simulink model "six_pulse_thyristor_based_rectifier"  (R2026b)
settings: Solver=ode23tb  StopTime=param.sim.simlength  FixedStep=param.glb_time.tc  MaxStep=param.glb_time.tc  EnableMultiTasking=on
values from neighbouring files (symbols this model uses):
  param = struct()    [init_model.m]    (also in init_model_legacy.m = add_template_extras(param, options))
undefined symbols (not defined in the file or in its folder): magnitude
libraries: fl_lib x168, nesl_utility x52, ee_lib x8, thyristor_rr_lib x6, first_harmonic_tracker x3, three_phase_voltage_with_frt_emulator x1
(part 1 of 4)
settings Model: Creator=LTNBDA  LastModifiedBy=d.bagnara
settings SolverCC: SolverResetMethod=Robust  ZeroCrossAlgorithm=Adaptive  ZeroCrossControl=EnableAll
settings DataIOCC: LimitDataPoints=on  MaxDataPoints=1  ReturnWorkspaceOutputs=off  SaveFormat=Array  SignalLoggingSaveFormat=ModelDataLogs
settings OptimizationCC: EfficientMapNaN2IntZero=off  LifeSpan=inf  MemsetInitFltsAndDblsToZero=off
settings DebuggingCC: ArithmeticOperatorsInVariantConditions=warning  FcnCallInpInsideContextMsg=warning  MergeDetectMultiDrivingBlocksExec=none  MultiTaskCondExecSysMsg=none  MultiTaskDSMMsg=warning  SFNoUnconditionalDefaultTransitionDiag=warning  SFUnexpectedBacktrackingDiag=warning  SaveWithParameterizedLinksMsg=none  SignalResolutionControl=TryResolveAllWithWarning  SolverPrmCheckMsg=warning  StateNameClashWarn=warning
settings HardwareCC: ProdEndianess=Unspecified  ProdEqTarget=off  ProdHWDeviceType=Generic->64-bit Embedded Processor (LP64)  ProdIntDivRoundTo=Undefined  ProdLargestAtomicFloat=None  TargetEndianess=LittleEndian  TargetHWDeviceType=MATLAB Host  TargetIntDivRoundTo=Zero  TargetLongLongMode=on
settings ModelReferenceCC: PropagateSignalLabelsOutOfModel=off
settings SFSimCC: CustomCodeUndefinedFunction=UseInterfaceOnly  SimUseLocalCustomCode=off
settings SFSimCC: SimCustomHeaderCode=|
  | #include "math_f.h"
  | #include "mavgflt.h"
  | #include "mavgflt_simulink.h"
  | #include "bemf_obsv.h"
  | #include "bemf_obsv_simulink.h"
  | #include "bemf_obsv_load_est.h"
  | #include "bemf_obsv_load_est_simulink.h"
  | #include "dqvector_pi.h"
  | #include "dqvector_pi_simulink.h"
  | #include "sv_pwm_simulink.h"
  | #include "sv_pwm.h"
  | #include "six_pulse_rect.h"
  | #include "twelve_pulse_rect.h"
  | #include "first_harmonic_tracker.h"
  | #include "first_harmonic_tracker_simulink.h"
  | #include "dqpll_thyr.h"
  | #include "dqpll_thyr_simulink.h"
  | #include "dqpll_grid.h"
  | #include "dqpll_grid_simulink.h"
settings SFSimCC: SimUserIncludeDirs=|
  | include
  | src
settings SFSimCC: SimUserSources=|
  | "mavgflt_simulink.c"
  | "mavgflt.c"
  | "bemf_obsv_simulink.c"
  | "bemf_obsv.c"
  | "bemf_obsv_load_est_simulink.c"
  | "bemf_obsv_load_est.c"
  | "dqvector_pi.c"
  | "dqvector_pi_simulink.c"
  | "sv_pwm_simulink.c"
  | "sv_pwm.c"
  | "six_pulse_rect.c"
  | "twelve_pulse_rect.c"
  | "first_harmonic_tracker_simulink.c"
  | "first_harmonic_tracker.c"
  | "dqpll_thyr_simulink.c"
  | "dqpll_thyr.c"
  | "dqpll_grid_simulink.c"
  | "dqpll_grid.c"
settings RTWCC: RTWUseLocalCustomCode=off
settings CodeAppCC: StateflowObjectComments=on
settings GRTTargetCC: CombineOutputUpdateFcns=off  GRTInterface=on  TargetLangStandard=C89/C90 (ANSI)
settings ConfigComp: CovExternalEMLEnable=off  CovSaveCumulativeToWorkspaceVar=on  CovSaveSingleToWorkspaceVar=on
settings SimscapeCC: SimscapeNormalizeSystem=off  SimscapeUseEnergyAccounting=off

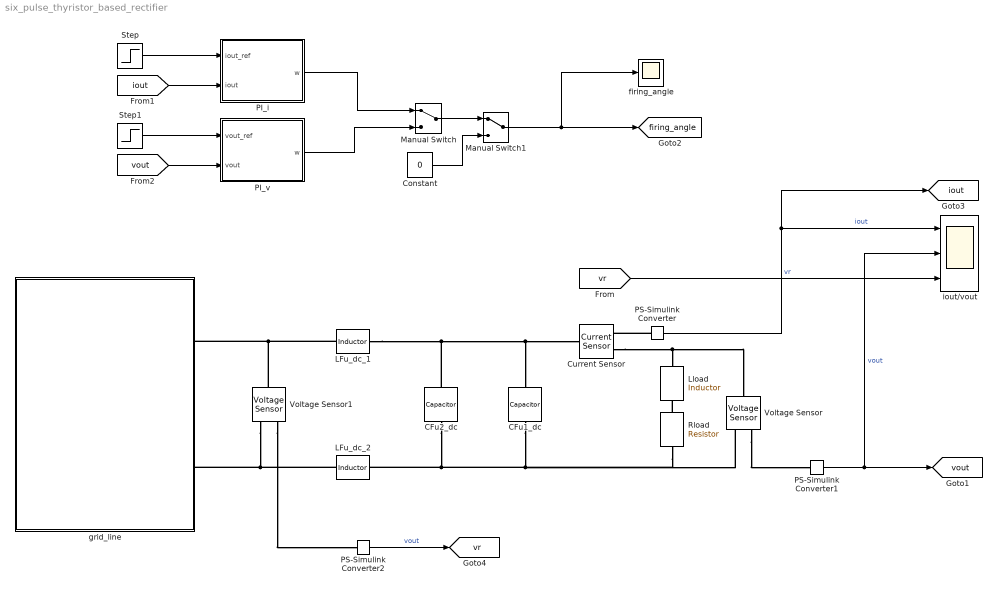
== system six_pulse_thyristor_based_rectifier ==
  CFu1_dc : fl_lib/Electrical/Electrical Elements/Capacitor  c=param.rect.hw.CFu1_dc F  r=param.rect.hw.RCFu1_dc Ohm  g=0 1/Ohm  i_specify=off  i_priority=None  i=0 A  i_nominal_specify=off  i_nominal_value=1  i_nominal_unit=A  v_specify=off  v_priority=None  v=0 V  v_nominal_specify=off  v_nominal_value=1  v_nominal_unit=V  vc_specify=off  vc_priority=High  vc=0 V  vc_nominal_specify=off  vc_nominal_value=1  vc_nominal_unit=V
  CFu2_dc : fl_lib/Electrical/Electrical Elements/Capacitor  c=param.rect.hw.CFu2_dc F  r=param.rect.hw.RCFu2_dc Ohm  g=0 1/Ohm  i_specify=off  i_priority=None  i=0 A  i_nominal_specify=off  i_nominal_value=1  i_nominal_unit=A  v_specify=off  v_priority=None  v=0 V  v_nominal_specify=off  v_nominal_value=1  v_nominal_unit=V  vc_specify=off  vc_priority=High  vc=0 V  vc_nominal_specify=off  vc_nominal_value=1  vc_nominal_unit=V
  Constant : Constant  Value=0
  Current Sensor : fl_lib/Electrical/Electrical Sensors/Current Sensor
  LFu_dc_1 : fl_lib/Electrical/Electrical Elements/Inductor  l=param.rect.hw.LFu_dc/2 H  r=param.rect.hw.RLFu_dc/2 Ohm  g=1e-9 1/Ohm  i_specify=off  i_priority=None  i=0 A  i_nominal_specify=off  i_nominal_value=1  i_nominal_unit=A  v_specify=off  v_priority=None  v=0 V  v_nominal_specify=off  v_nominal_value=1  v_nominal_unit=V  i_L_specify=off  i_L_priority=High  i_L=0 A  i_L_nominal_specify=off  i_L_nominal_value=1  i_L_nominal_unit=A
  LFu_dc_2 : fl_lib/Electrical/Electrical Elements/Inductor  l=param.rect.hw.LFu_dc/2 H  r=param.rect.hw.RLFu_dc/2 Ohm  g=1e-9 1/Ohm  i_specify=off  i_priority=None  i=0 A  i_nominal_specify=off  i_nominal_value=1  i_nominal_unit=A  v_specify=off  v_priority=None  v=0 V  v_nominal_specify=off  v_nominal_value=1  v_nominal_unit=V  i_L_specify=off  i_L_priority=High  i_L=0 A  i_L_nominal_specify=off  i_L_nominal_value=1  i_L_nominal_unit=A
  Lload : fl_lib/Electrical/Electrical Elements/Inductor  l=param.load.L H  r=0 Ohm  g=1e-9 1/Ohm  i_specify=off  i_priority=None  i=0 A  i_nominal_specify=off  i_nominal_value=1  i_nominal_unit=A  v_specify=off  v_priority=None  v=0 V  v_nominal_specify=off  v_nominal_value=1  v_nominal_unit=V  i_L_specify=off  i_L_priority=High  i_L=0 A  i_L_nominal_specify=off  i_L_nominal_value=1  i_L_nominal_unit=A
  Manual Switch : ManualSwitch
  Manual Switch1 : ManualSwitch
  PI_i : Subsystem
  PI_v : Subsystem
  PS-Simulink Converter : nesl_utility/PS-Simulink Converter  PhysicalDomain=network_engine_domain  SubClassName=ps_output  LeftPortType=input  RightPortType=output  PseudoPeriodic=off  Frequencies=[]  VectorFormat=1-D array  Unit=A  AffineConversion=off
  PS-Simulink Converter1 : nesl_utility/PS-Simulink Converter  PhysicalDomain=network_engine_domain  SubClassName=ps_output  LeftPortType=input  RightPortType=output  PseudoPeriodic=off  Frequencies=[]  VectorFormat=1-D array  Unit=V  AffineConversion=on
  PS-Simulink Converter2 : nesl_utility/PS-Simulink Converter  PhysicalDomain=network_engine_domain  SubClassName=ps_output  LeftPortType=input  RightPortType=output  PseudoPeriodic=off  Frequencies=[]  VectorFormat=1-D array  Unit=V  AffineConversion=on
  Rload : fl_lib/Electrical/Electrical Elements/Resistor  R=param.load.R Ohm  i_specify=off  i_priority=None  i=0 A  i_nominal_specify=off  i_nominal_value=1  i_nominal_unit=A  v_specify=off  v_priority=None  v=0 V  v_nominal_specify=off  v_nominal_value=1  v_nominal_unit=V
  Step : Step  Time=param.rect.ctrl.t_iref_step  InitialValue=param.rect.ctrl.iref_1/param.meas.I_FS  FinalValue=param.rect.ctrl.iref_2/param.meas.I_FS  SampleTime=0
  Step1 : Step  Time=0  FinalValue=param.rect.ctrl.vref/param.meas.V_FS  SampleTime=0
  Voltage Sensor : fl_lib/Electrical/Electrical Sensors/Voltage Sensor
  Voltage Sensor1 : fl_lib/Electrical/Electrical Sensors/Voltage Sensor
  firing_angle : Scope
      settings: ActiveDisplayYMinimum=-0.39269908169872403  ActiveDisplayYMaximum=3.5342917352885173  DataLoggingVariableName=ScopeData5
  grid_line : Subsystem
  iout/vout : Scope  NumInputPorts=3
      settings: ActiveDisplayYMinimum=-22.431866208860185  ActiveDisplayYMaximum=201.8867958797417  DataLoggingVariableName=ScopeData10
  tag scope: firing_angle=global, iout=global, vout=global, vr=global
  wires:
  PS-Simulink Converter/1 -> [iout], iout/vout/1  "iout"
  Step/1 -> PI_i/1(iout_ref)
  PS-Simulink Converter1/1 -> [vout], iout/vout/2  "vout"
  [iout] -> PI_i/2(iout)
  [vout] -> PI_v/2(vout)
  Step1/1 -> PI_v/1(vout_ref)
  PI_i/1(w) -> Manual Switch/1
  PI_v/1(w) -> Manual Switch/2
  Manual Switch/1 -> Manual Switch1/1
  Manual Switch1/1 -> [firing_angle], firing_angle/1
  Constant/1 -> Manual Switch1/2
  PS-Simulink Converter2/1 -> [vr]  "vout"
  [vr] -> iout/vout/3  "vr"
  connections:
  LFu_dc_1/RConn1 -- CFu2_dc/LConn1 -- Current Sensor/LConn1 -- CFu1_dc/LConn1
  CFu1_dc/RConn1 -- LFu_dc_2/LConn1 -- CFu2_dc/RConn1 -- Voltage Sensor/RConn2 -- Rload/RConn1
  LFu_dc_2/RConn1 -- Voltage Sensor1/RConn2 -- grid_line/RConn2
  LFu_dc_1/LConn1 -- Voltage Sensor1/LConn1 -- grid_line/RConn1
  Rload/LConn1 -- Lload/RConn1
  PS-Simulink Converter/LConn1 -- Current Sensor/RConn1
  Current Sensor/RConn2 -- Voltage Sensor/LConn1 -- Lload/LConn1
  Voltage Sensor/RConn1 -- PS-Simulink Converter1/LConn1
  Voltage Sensor1/RConn1 -- PS-Simulink Converter2/LConn1

== system six_pulse_thyristor_based_rectifier/PI_i ==
  iout_ref : Inport
  iout : Inport  Port=2
  1/Ti : Gain  Gain=param.rect.ctrl.pi_i.kp  SaturateOnIntegerOverflow=on  OutDataTypeStr=Inherit: Same as input  ParamDataTypeStr=Inherit: Same as input
  1/Ti2 : Gain  Gain=1/param.meas.I_FS  SaturateOnIntegerOverflow=on  OutDataTypeStr=Inherit: Same as input  ParamDataTypeStr=Inherit: Same as input
  Saturation : Saturate  UpperLimit=param.rect.ctrl.alpha_max  LowerLimit=param.rect.ctrl.alpha_min
  Saturation1 : Saturate  UpperLimit=param.rect.ctrl.u_max  LowerLimit=param.rect.ctrl.u_min
  Sum1 : Sum  Inputs=+++  SaturateOnIntegerOverflow=on
  Sum2 : Sum  Inputs=+-  SaturateOnIntegerOverflow=on
  Sum3 : Sum  Inputs=-+  SaturateOnIntegerOverflow=on
  Trigonometric Function : Trigonometry  Operator=acos
  Unit Delay1 : UnitDelay  SampleTime=param.glb_time.ts_rect
  Unit Delay4 : UnitDelay  SampleTime=param.glb_time.ts_rect
  kp : Gain  Gain=param.rect.ctrl.pi_i.ki*param.glb_time.ts_rect  SaturateOnIntegerOverflow=on  OutDataTypeStr=Inherit: Same as input  ParamDataTypeStr=Inherit: Same as input
  tracking_current : Scope  NumInputPorts=2
      settings: ActiveDisplayYMinimum=-0.16727670721082677  ActiveDisplayYMaximum=1.5054903648974411  DataLoggingVariableName=ScopeData7
  w : Outport  VectorParamsAs1DForOutWhenUnconnected=off
  wires:
  Sum2/1 -> 1/Ti/1, kp/1
  kp/1 -> Sum1/2
  1/Ti/1 -> Sum3/1, Sum1/1
  Unit Delay4/1 -> Sum1/3
  Sum3/1 -> Unit Delay4/1
  Sum1/1 -> Saturation1/1
  Saturation/1 -> Unit Delay1/1
  iout/1 -> 1/Ti2/1
  iout_ref/1 -> tracking_current/1, Sum2/1  "i_out_ref"
  1/Ti2/1 -> Sum2/2, tracking_current/2  "i_out"
  Unit Delay1/1 -> w/1
  Saturation1/1 -> Sum3/2, Trigonometric Function/1
  Trigonometric Function/1 -> Saturation/1

== system six_pulse_thyristor_based_rectifier/PI_v ==
  vout_ref : Inport
  vout : Inport  Port=2
  1/Ti : Gain  Gain=param.rect.ctrl.pi_v.kp  SaturateOnIntegerOverflow=on  OutDataTypeStr=Inherit: Same as input  ParamDataTypeStr=Inherit: Same as input
  1/Ti2 : Gain  Gain=1/param.meas.V_FS  SaturateOnIntegerOverflow=on  OutDataTypeStr=Inherit: Same as input  ParamDataTypeStr=Inherit: Same as input
  Saturation : Saturate  UpperLimit=param.rect.ctrl.alpha_max  LowerLimit=param.rect.ctrl.alpha_min
  Saturation1 : Saturate  UpperLimit=param.rect.ctrl.u_max  LowerLimit=param.rect.ctrl.u_min
  Sum1 : Sum  Inputs=+++  SaturateOnIntegerOverflow=on
  Sum2 : Sum  Inputs=+-  SaturateOnIntegerOverflow=on
  Sum3 : Sum  Inputs=-+  SaturateOnIntegerOverflow=on
  Trigonometric Function : Trigonometry  Operator=acos
  Unit Delay1 : UnitDelay  SampleTime=param.glb_time.ts_rect
  Unit Delay4 : UnitDelay  SampleTime=param.glb_time.ts_rect
  kp : Gain  Gain=param.rect.ctrl.pi_v.ki*param.glb_time.ts_rect  SaturateOnIntegerOverflow=on  OutDataTypeStr=Inherit: Same as input  ParamDataTypeStr=Inherit: Same as input
  w : Outport  VectorParamsAs1DForOutWhenUnconnected=off
  wires:
  Trigonometric Function/1 -> Saturation/1
  Saturation1/1 -> Trigonometric Function/1, Sum3/2
  Unit Delay1/1 -> w/1
  1/Ti2/1 -> Sum2/2
  vout_ref/1 -> Sum2/1
  vout/1 -> 1/Ti2/1
  Saturation/1 -> Unit Delay1/1
  Sum1/1 -> Saturation1/1
  Sum3/1 -> Unit Delay4/1
  Unit Delay4/1 -> Sum1/3
  1/Ti/1 -> Sum1/1, Sum3/1
  kp/1 -> Sum1/2
  Sum2/1 -> kp/1, 1/Ti/1

== system six_pulse_thyristor_based_rectifier/grid_line ==
  Grid : Subsystem
  six_pulse rectifier : Subsystem
  DC+ : PMIOPort  Side=Right
  DC- : PMIOPort  Port=2  Side=Right
  connections:
  six_pulse rectifier/RConn1 -- DC+/RConn1
  Grid/RConn1 -- six_pulse rectifier/LConn1
  six_pulse rectifier/RConn2 -- DC-/RConn1

== system six_pulse_thyristor_based_rectifier/grid_line/Grid ==
  Dyg_TR : Subsystem
  grid_emulator : Subsystem
  pwr-measurement : Subsystem
  u_grid : PMIOPort  Side=Right
  connections:
  Dyg_TR/LConn2 -- grid_emulator/RConn2
  Dyg_TR/LConn1 -- grid_emulator/RConn1
  Dyg_TR/LConn3 -- grid_emulator/RConn3
  Dyg_TR/RConn1 -- u_grid/RConn1

== system six_pulse_thyristor_based_rectifier/grid_line/six_pulse rectifier ==
  BR2 : Subsystem
  C-caller ctrl : Subsystem
  Inductor : fl_lib/Electrical/Electrical Elements/Inductor  l=param.rect.hw.Lac H  r=0 Ohm  g=1e-9 1/Ohm  i_specify=off  i_priority=None  i=0 A  i_nominal_specify=off  i_nominal_value=1  i_nominal_unit=A  v_specify=off  v_priority=None  v=0 V  v_nominal_specify=off  v_nominal_value=1  v_nominal_unit=V  i_L_specify=off  i_L_priority=High  i_L=0 A  i_L_nominal_specify=off  i_L_nominal_value=1  i_L_nominal_unit=A
  Inductor1 : fl_lib/Electrical/Electrical Elements/Inductor  l=param.rect.hw.Lac H  r=0 Ohm  g=1e-9 1/Ohm  i_specify=off  i_priority=None  i=0 A  i_nominal_specify=off  i_nominal_value=1  i_nominal_unit=A  v_specify=off  v_priority=None  v=0 V  v_nominal_specify=off  v_nominal_value=1  v_nominal_unit=V  i_L_specify=off  i_L_priority=High  i_L=0 A  i_L_nominal_specify=off  i_L_nominal_value=1  i_L_nominal_unit=A
  Inductor2 : fl_lib/Electrical/Electrical Elements/Inductor  l=param.rect.hw.Lac H  r=0 Ohm  g=1e-9 1/Ohm  i_specify=off  i_priority=None  i=0 A  i_nominal_specify=off  i_nominal_value=1  i_nominal_unit=A  v_specify=off  v_priority=None  v=0 V  v_nominal_specify=off  v_nominal_value=1  v_nominal_unit=V  i_L_specify=off  i_L_priority=High  i_L=0 A  i_L_nominal_specify=off  i_L_nominal_value=1  i_L_nominal_unit=A
  Phase Splitter2 : ee_lib/Connectors & References/Phase Splitter
  Scope2 : Scope
      settings: SampleTime=param.glb_time.ts_rect  ActiveDisplayYMinimum=-0.78504431247711159  ActiveDisplayYMaximum=7.0653988122940063
  Step : Step  Time=param.rect.ctrl.t_pulse_release  InitialValue=1  FinalValue=0  SampleTime=param.glb_time.ts_rect
  pll : Subsystem
  ui/grid : Scope  NumInputPorts=2
      settings: ActiveDisplayYMinimum=-5.4212636300708823  ActiveDisplayYMaximum=7.6356213899946326
  voltage_measure1 : Subsystem
  voltage_measure2 : Subsystem
  DC+ : PMIOPort  Side=Right
  grid_line : PMIOPort  Port=2  Side=Left
  DC- : PMIOPort  Port=3  Side=Right
  wires:
  voltage_measure2/1(vabc_grid) -> ui/grid/1
  Step/1 -> C-caller ctrl/3(Block)
  pll/1(grid_phase_hat) -> Scope2/1, C-caller ctrl/2(wt)
  [firing_angle] -> C-caller ctrl/1(alpha)
  voltage_measure2/2(iabc_grid) -> ui/grid/2
  C-caller ctrl/1(firing_cmds) -> BR2/1(firing_cmds)
  connections:
  voltage_measure2/RConn1 -- BR2/RConn1
  grid_line/RConn1 -- Phase Splitter2/LConn1
  voltage_measure1/LConn2 -- Inductor1/RConn1 -- voltage_measure2/LConn2
  voltage_measure1/LConn3 -- Inductor2/RConn1 -- voltage_measure2/LConn3
  BR2/LConn2 -- DC-/RConn1
  voltage_measure2/RConn3 -- BR2/RConn3
  voltage_measure1/LConn1 -- Inductor/RConn1 -- voltage_measure2/LConn1
  voltage_measure2/RConn2 -- BR2/RConn2
  BR2/LConn1 -- DC+/RConn1
  Phase Splitter2/RConn1 -- Inductor/LConn1
  Phase Splitter2/RConn2 -- Inductor1/LConn1
  Phase Splitter2/RConn3 -- Inductor2/LConn1

== system six_pulse_thyristor_based_rectifier/grid_line/Grid/Dyg_TR ==
  Electrical Reference : fl_lib/Electrical/Electrical Elements/Electrical Reference
  PS Terminator : fl_lib/Physical Signals/Sinks/PS Terminator
  PS Terminator1 : fl_lib/Physical Signals/Sinks/PS Terminator
  PS Terminator2 : fl_lib/Physical Signals/Sinks/PS Terminator
  Phase Splitter : ee_lib/Connectors & References/Phase Splitter
  configurable_trafo : SimscapeComponentBlock  Description=Configurable transformer: one or two three-phase primaries (star or delta), secondary three-phase (star or delta, any clock number) or single-phase (turns distribution ws) on a three-limb core. Component configurable_transformer.configurable_transformer (pwr-control/library, foundation/electrical_machines/+configurable_transformer).  SourceFile=configurable_transformer.configurable_transformer  ComponentPath=configurable_transformer.configurable_transformer  ComponentVariants="[\"configurable_transformer.configurable_transformer\"]"  ComponentVariantNames="[\"configurable_transformer\"]"  ClassName=configurable_transformer  SchemaVersion=1  primaries=configurable_transformer.n_primaries.one  conn1=configurable_transformer.connection.delta  conn2=configurable_transformer.connection.star  clock2=param.grid.trafo.clock2  secondary=configurable_transformer.secondary_winding.star  clock3=param.grid.trafo.clock3  ws=[1, -1, 0]  Sr=param.grid.trafo.Sr A*V  V1=param.grid.trafo.V1 V  V2=param.grid.trafo.V2 V  V3=param.grid.trafo.V3 V  fr=param.grid.trafo.fr Hz  r1=param.grid.trafo.r1  l1=param.grid.trafo.l1  r2=param.grid.trafo.r2  l2=param.grid.trafo.l2  r3=param.grid.trafo.r3  l3=param.grid.trafo.l3  lm=param.grid.trafo.lm  lm0=param.grid.trafo.lm0  rfe=param.grid.trafo.rfe  i1a_specify=off  i1a_priority=None  i1a=0 A  i1a_nominal_specify=off  i1a_nominal_value=1  i1a_nominal_unit=A  i1b_specify=off  i1b_priority=None  i1b=0 A  i1b_nominal_specify=off  i1b_nominal_value=1  i1b_nominal_unit=A  i1c_specify=off  i1c_priority=None  i1c=0 A  i1c_nominal_specify=off  i1c_nominal_value=1  i1c_nominal_unit=A  i2a_specify=off  i2a_priority=None  i2a=0 A  i2a_nominal_specify=off  i2a_nominal_value=1  i2a_nominal_unit=A  i2b_specify=off  i2b_priority=None  i2b=0 A  i2b_nominal_specify=off  i2b_nominal_value=1  i2b_nominal_unit=A  i2c_specify=off  i2c_priority=None  i2c=0 A  i2c_nominal_specify=off  i2c_nominal_value=1  i2c_nominal_unit=A  i3a_specify=off  i3a_priority=None  i3a=0 A  i3a_nominal_specify=off  i3a_nominal_value=1  i3a_nominal_unit=A  i3b_specify=off  i3b_priority=None  i3b=0 A  i3b_nominal_specify=off  i3b_nominal_value=1  i3b_nominal_unit=A  i3c_specify=off  i3c_priority=None  i3c=0 A  i3c_nominal_specify=off  i3c_nominal_value=1  i3c_nominal_unit=A  i3_specify=off  i3_priority=None  i3=0 A  i3_nominal_specify=off  i3_nominal_value=1  i3_nominal_unit=A
      settings: CopyFcn=simscape.sscblock.internal.componentBlockCallback(gcbh,'COPY')  PreCopyFcn=simscape.sscblock.internal.componentBlockCallback(gcbh,'PRECOPY')  PreDeleteFcn=simscape.sscblock.internal.componentBlockCallback(gcbh,'PREDELETE')
      mask Type: Configurable Transformer
  ui_meas : Subsystem
  u1_a : PMIOPort  Side=Left
  u1_b : PMIOPort  Port=2  Side=Left
  u1_c : PMIOPort  Port=3  Side=Left
  u2_abc : PMIOPort  Port=4  Side=Right
  connections:
  configurable_trafo/LConn1 -- u1_a/RConn1
  configurable_trafo/LConn2 -- u1_b/RConn1
  configurable_trafo/LConn3 -- u1_c/RConn1
  configurable_trafo/RConn4 -- Electrical Reference/LConn1
  u2_abc/RConn1 -- Phase Splitter/LConn1
  PS Terminator/LConn1 -- configurable_trafo/RConn5
  PS Terminator1/LConn1 -- configurable_trafo/RConn6
  configurable_trafo/RConn7 -- PS Terminator2/LConn1
  ui_meas/LConn2 -- configurable_trafo/RConn2
  ui_meas/LConn1 -- configurable_trafo/RConn1
  ui_meas/LConn3 -- configurable_trafo/RConn3
  Phase Splitter/RConn3 -- ui_meas/RConn3
  Phase Splitter/RConn2 -- ui_meas/RConn2
  Phase Splitter/RConn1 -- ui_meas/RConn1

== system six_pulse_thyristor_based_rectifier/grid_line/Grid/grid_emulator ==
  Bus Selector : BusSelector  OutputSignals=ua_grid_emu,ub_grid_emu,uc_grid_emu
  Bus Selector1 : BusSelector  OutputSignals=gamma_grid_emulator,omega_grid_emulator
  Controlled Voltage Source : fl_lib/Electrical/Electrical Sources/Controlled Voltage Source
  Controlled Voltage Source1 : fl_lib/Electrical/Electrical Sources/Controlled Voltage Source
  Controlled Voltage Source2 : fl_lib/Electrical/Electrical Sources/Controlled Voltage Source
  Electrical Reference : fl_lib/Electrical/Electrical Elements/Electrical Reference
  Simulink-PS Converter : nesl_utility/Simulink-PS Converter  PhysicalDomain=network_engine_domain  SubClassName=ps_input  LeftPortType=input  RightPortType=output  PseudoPeriodic=off  Frequencies=[]  NoiseDistribution=none  NoiseParameters=[]  Unit=V  AffineConversion=on  FilteringAndDerivatives=provide  SimscapeFilterOrder=1  InputFilterTimeConstant=0.001  UdotUserProvided=0
  Simulink-PS Converter1 : nesl_utility/Simulink-PS Converter  PhysicalDomain=network_engine_domain  SubClassName=ps_input  LeftPortType=input  RightPortType=output  PseudoPeriodic=off  Frequencies=[]  NoiseDistribution=none  NoiseParameters=[]  Unit=V  AffineConversion=on  FilteringAndDerivatives=provide  SimscapeFilterOrder=1  InputFilterTimeConstant=0.001  UdotUserProvided=0
  Simulink-PS Converter2 : nesl_utility/Simulink-PS Converter  PhysicalDomain=network_engine_domain  SubClassName=ps_input  LeftPortType=input  RightPortType=output  PseudoPeriodic=off  Frequencies=[]  NoiseDistribution=none  NoiseParameters=[]  Unit=V  AffineConversion=on  FilteringAndDerivatives=provide  SimscapeFilterOrder=1  InputFilterTimeConstant=0.001  UdotUserProvided=0
  Solver Configuration : nesl_utility/Solver Configuration  PhysicalDomain=network_engine_domain  SubClassName=solver  LeftPortType=input  RightPortType=generic  Tones=[]  Harmonics=[]  SimulateNoise=off  Profile=off  UseLocalSampling=off  EnableSwitchedLinearOptims=on  FrequencyDomain=off  UseCCode=off  RelTol=0.001  AbsTol=1e-06  MinStep=1e-09  ToWorkspace=off  RevertToSquareIcSolve=off  NumHomotopyIterations=100  PhasorMode=off  PhasorModeNumHarmonics=1  ConsistencySolver=NEWTON_FTOL  CanonicalOrdering=UNORDERED  OptimizeIntermediates=UNOPTIMIZED  MulticoreSolverChoice=BACKWARD_EULER  IndexReductionMethod=DerivativeReplacement  DoDC=on  ResidualTolerance=1e-4  ConsistencyTolSource=GLOBAL  ConsistencyAbsTol=0.001  ConsistencyRelTol=0.001  ConsistencyTolFactor=0.001  UseLocalSolver=on  LocalSolverChoice=NE_TRAPEZOIDAL_ADVANCER  ResolveIndetEquations=on  FunctionEvalNumThread=1  LocalSolverSampleTime=param.glb_time.tc  DoFixedCost=on  MaxNonlinIter=param.sim.nonlinear_iterations  MaxModeIter=2  ComputeImpulses=off  ImpulseIterations=2  LinearAlgebra=auto  LinearAlgebraNumThread=0  EquationFormulation=NE_TIME_EF  DelaysMemoryBudget=1024  AutomaticFiltering=on  FilteringTimeConstant=0.001  PartitionStorageMethod=AS_NEEDED  PartitionMemoryBudget=1024  PartitionMethod=BALANCED  MultibodyUseLocalSolver=off  MultibodyLocalSolverChoice=ODE1  MultibodyLocalSolverSampleTime=0.001
  three_phase_voltage_source_with_frt_emulator : three_phase_voltage_with_frt_emulator/three_phase_voltage_source_with_frt_emulator  nominal_frequency_m=param.grid.emu.fgrid_nom  nominal_voltage_m=param.grid.emu.us_nom  Vemu_ref_norm_m=param.grid.emu.Vemu_ref_norm  vp_xi_pu_m=param.grid.emu.up_xi_pu_ref  vp_eta_pu_m=param.grid.emu.up_eta_pu_ref  vn_xi_pu_m=param.grid.emu.un_xi_pu_ref  vn_eta_pu_m=param.grid.emu.un_eta_pu_ref  Am=param.grid.emu.sof_50Hz.A  Bm=param.grid.emu.sof_50Hz.B  Cm=param.grid.emu.sof_50Hz.C  enable_frt_1_m=param.grid.frt.enable_frt_1  enable_frt_2_m=param.grid.frt.enable_frt_2  start_time_LVRT_m=param.grid.frt.start_time_LVRT  end_time_LVRT_m=param.grid.frt.end_time_LVRT  deepPOSxi_m=param.grid.frt.deepPOSxi  deepPOSeta_m=param.grid.frt.deepPOSeta  deepNEGxi_m=param.grid.frt.deepNEGxi  deepNEGeta_m=param.grid.frt.deepNEGeta  Amplitude_U_m=param.grid.frt.Amplitude_U  Amplitude_V_m=param.grid.frt.Amplitude_V  Amplitude_W_m=param.grid.frt.Amplitude_W  t_ramp_m=param.grid.frt.t_ramp  Phase_shift_m=param.grid.frt.Phase_shift
  threephase_vi_measures : Subsystem
  u1 : PMIOPort  Side=Right
  u2 : PMIOPort  Port=2  Side=Right
  u3 : PMIOPort  Port=3  Side=Right
  tag scope: phase_grid_emulator=global, pulsation_grid_emulator=global
  wires:
  Bus Selector1/2 -> [pulsation_grid_emulator]  "<omega_grid_emulator>"
  Bus Selector1/1 -> [phase_grid_emulator]  "<gamma_grid_emulator>"
  Bus Selector/2 -> Simulink-PS Converter1/1  "<ub_grid_emu>"
  Bus Selector/3 -> Simulink-PS Converter2/1  "<uc_grid_emu>"
  three_phase_voltage_source_with_frt_emulator/1 -> Bus Selector1/1, Bus Selector/1
  Bus Selector/1 -> Simulink-PS Converter/1  "<ua_grid_emu>"
  connections:
  Simulink-PS Converter/RConn1 -- Controlled Voltage Source/RConn1
  Simulink-PS Converter1/RConn1 -- Controlled Voltage Source1/RConn1
  Simulink-PS Converter2/RConn1 -- Controlled Voltage Source2/RConn1
  Controlled Voltage Source/RConn2 -- Controlled Voltage Source1/RConn2 -- Solver Configuration/RConn1 -- Electrical Reference/LConn1 -- Controlled Voltage Source2/RConn2
  u1/RConn1 -- threephase_vi_measures/RConn1
  u2/RConn1 -- threephase_vi_measures/RConn2
  u3/RConn1 -- threephase_vi_measures/RConn3
  Controlled Voltage Source/LConn1 -- threephase_vi_measures/LConn1
  Controlled Voltage Source1/LConn1 -- threephase_vi_measures/LConn2
  Controlled Voltage Source2/LConn1 -- threephase_vi_measures/LConn3

== system six_pulse_thyristor_based_rectifier/grid_line/Grid/pwr-measurement ==
  THD : Subsystem
  power meter iec mfunc : Subsystem
  ui/line : Scope  NumInputPorts=2
      settings: SampleTime=param.glb_time.ts_rect  ActiveDisplayYMinimum=-245.71044409465458  ActiveDisplayYMaximum=198.75905970575923
  wires:
  [i_abc_line] -> ui/line/1
  [u_abc_line] -> ui/line/2

== system six_pulse_thyristor_based_rectifier/grid_line/six_pulse rectifier/BR2 ==
  firing_cmds : Inport
  Bus Creator : BusCreator  Inputs=3
  Selector : Selector  InputPortWidth=6  IndexOptions=Index vector (dialog)  Indices=1  OutputSizes=1  RuntimeRangeChecks=off
  Selector1 : Selector  InputPortWidth=6  IndexOptions=Index vector (dialog)  Indices=1  OutputSizes=1  RuntimeRangeChecks=off
  Selector2 : Selector  InputPortWidth=6  IndexOptions=Index vector (dialog)  Indices=1  OutputSizes=1  RuntimeRangeChecks=off
  TR_id_rr : Scope  NumInputPorts=4
      settings: ActiveDisplayYMinimum=-1.4999999999999996  ActiveDisplayYMaximum=13.5  DataLoggingVariableName=ScopeData6
  To Workspace : ToWorkspace  VariableName=thyristor_data  SaveFormat=Structure With Time  SampleTime=param.glb_time.tc
      settings: MaxDataPoints=param.glb_time.Nc
  rc_snubber_current_rms : Scope
      settings: ActiveDisplayYMinimum=-0.019484294170770761  ActiveDisplayYMaximum=0.17535887386370427  DataLoggingVariableName=ScopeData8
  rms : Subsystem
  ssc_thyristor_bridge : Subsystem  mask{Vf_m=param.rect.thy.Vf, Ron_m=param.rect.thy.Ron, Goff_m=param.rect.thy.Goff, forward_voltage_threshold_m=param.rect.thy.Vth, Vgt_m=param.rect.thy.Vgt, latching_current_m=param.rect.thy.Il, holding_current_m=param.rect.thy.Ih, carrier_lifetime_m=param.rect.thy.tau, charge_cross_time_constant_m=param.rect.thy.Tm, residual_charge_threshold_m=param.rect.thy.Qth, circuit_commutated_turn_off_time_m=param.rect.thy.tq, t_firing_strobe_m=param.glb_time.ts_rect, Rsnubber_m=param.rect.snubber.R, Csnubber_m=param.rect.snubber.C}
      mask prompts: Vf_m "Vt [V]"; Ron_m "rt [Ohm]"; Goff_m "Goff [1/Ohm]"; forward_voltage_threshold_m "Voltage Retrigger Threshold [V]"; Vgt_m "Vth [V]"; latching_current_m "latching current [A]"; holding_current_m "holding current [A]"; carrier_lifetime_m "carrier lifetime [s]"; charge_cross_time_constant_m "charge extraction time constant [s]"; residual_charge_threshold_m "residual charge threshold [C]"; circuit_commutated_turn_off_time_m "circuit commutated turn off time [s]"; t_firing_strobe_m "t_firing_strobe [s]"; Rsnubber_m "Rsnubber [Ohm]"; Csnubber_m "Csnubber [F]"
  DC+ : PMIOPort  Side=Left
  DC- : PMIOPort  Port=2  Side=Left
  phA : PMIOPort  Port=3  Side=Right
  phB : PMIOPort  Port=4  Side=Right
  phC : PMIOPort  Port=5  Side=Right
  wires:
  firing_cmds/1 -> Selector/1, TR_id_rr/1, ssc_thyristor_bridge/1(firing_cmds)
  ssc_thyristor_bridge/1(m_i) -> Selector1/1, TR_id_rr/2
  ssc_thyristor_bridge/2(m_u) -> Selector2/1, TR_id_rr/3
  Bus Creator/1 -> To Workspace/1
  ssc_thyristor_bridge/3(m_rc_i) -> TR_id_rr/4, rms/1(in)
  rms/1(out) -> rc_snubber_current_rms/1  "rc_snubber_current_rms"
  Selector/1 -> Bus Creator/1  "cmd_thyristor"
  Selector1/1 -> Bus Creator/2  "i_thyristor"
  Selector2/1 -> Bus Creator/3  "u_ak_thyristor"
  connections:
  DC+/RConn1 -- ssc_thyristor_bridge/LConn1
  DC-/RConn1 -- ssc_thyristor_bridge/LConn2
  phA/RConn1 -- ssc_thyristor_bridge/RConn1
  phB/RConn1 -- ssc_thyristor_bridge/RConn2
  phC/RConn1 -- ssc_thyristor_bridge/RConn3

== system six_pulse_thyristor_based_rectifier/grid_line/six_pulse rectifier/C-caller ctrl ==
  alpha : Inport  SampleTime=param.glb_time.tc
  wt : Inport  Port=2  SampleTime=param.glb_time.tc
  Block : Inport  Port=3  SampleTime=param.glb_time.tc
  Data Type Conversion1 : DataTypeConversion  OutDataTypeStr=single  SaturateOnIntegerOverflow=off  RndMeth=Floor
  Data Type Conversion2 : DataTypeConversion  OutDataTypeStr=single  SaturateOnIntegerOverflow=off  RndMeth=Floor
  Data Type Conversion4 : DataTypeConversion  OutDataTypeStr=int32  SaturateOnIntegerOverflow=off  RndMeth=Floor
  Zero-Order Hold1 : ZeroOrderHold  SampleTime=param.glb_time.ts_rect
  Zero-Order Hold2 : ZeroOrderHold  SampleTime=param.glb_time.ts_rect
  Zero-Order Hold3 : ZeroOrderHold  SampleTime=param.glb_time.ts_rect
  ccaller : CCaller  FunctionName=sprcProcessSimulink  PortSpecificationStruct="%)30     .    ( <   8    (     @         %    \"     0    !     0         %  0 \"0    $    _    07)G3F%M90  4&]R=$YA;64 4V-O<&4     26YD97@     5'EP90      4VEZ90      27-';&]B86P   X    P    !@    @    $          4    (     0    (    !         !   @!W=   #@   #     &    \"     0         !0    @    !     @    $         $  \" '=T   .    .     8    (    !          %    \"     $    %     0         0  ...(+2073 chars)"  SampleTime=param.glb_time.ts_rect
  pulses : Scope  NumInputPorts=4
      settings: SampleTime=param.glb_time.tc  ActiveDisplayYMinimum=-1.4999999999999996  ActiveDisplayYMaximum=13.5  DataLoggingVariableName=ScopeData2
  shift_level : Subsystem
  firing_cmds : Outport  SampleTime=param.glb_time.tc  InitialOutput=0  VectorParamsAs1DForOutWhenUnconnected=off
  wires:
  alpha/1 -> Data Type Conversion2/1
  wt/1 -> Data Type Conversion1/1
  Data Type Conversion2/1 -> Zero-Order Hold2/1
  Data Type Conversion1/1 -> Zero-Order Hold3/1
  Data Type Conversion4/1 -> Zero-Order Hold1/1
  Zero-Order Hold3/1 -> pulses/2, ccaller/1  "phase"
  Zero-Order Hold2/1 -> pulses/3, ccaller/2  "firing_angle"
  Zero-Order Hold1/1 -> ccaller/3
  Block/1 -> Data Type Conversion4/1
  shift_level/1(PY) -> firing_cmds/1, pulses/1  "p"
  ccaller/1 -> shift_level/1("PY ")
  [grid_voltage_filtered] -> pulses/4

== system six_pulse_thyristor_based_rectifier/grid_line/six_pulse rectifier/pll ==
  Bus Creator : BusCreator  Inputs=2
  Bus Selector : BusSelector  OutputSignals=phase_hat
  dqpll_thyr_ccaller : Subsystem
  dqpll_thyr_ccaller_s : Scope
      settings: ActiveDisplayYMinimum=-1.910201348364353  ActiveDisplayYMaximum=7.1920475736260414
  grid_phase_hats : Scope
      settings: ActiveDisplayYMinimum=-0.78537  ActiveDisplayYMaximum=7.06836  DataLoggingVariableName=ScopeData2
  pll_stageA : Subsystem
  pll_stageB : Subsystem
  grid_phase_hat : Outport
  wires:
  pll_stageA/1(Vgrid_a) -> pll_stageB/1(Vgrid_a)
  pll_stageA/2(Vgrid_b) -> pll_stageB/2(Vgrid_b)
  [vabc_grid_A] -> pll_stageA/1(ug)
  pll_stageB/1(wt_grid) -> Bus Creator/2  "grid_phase_hat_simulink"
  Bus Creator/1 -> grid_phase_hats/1
  dqpll_thyr_ccaller/1(m) -> dqpll_thyr_ccaller_s/1, Bus Selector/1
  Bus Selector/1 -> Bus Creator/1, grid_phase_hat/1  "<phase_hat>"

== system six_pulse_thyristor_based_rectifier/grid_line/six_pulse rectifier/voltage_measure1 ==
  Gain4 : Gain  Gain=1/3
  Gain5 : Gain  Gain=1/3
  Gain6 : Gain  Gain=1/3
  Mux : Mux  Inputs=3
  PS-Simulink Converter : nesl_utility/PS-Simulink Converter  PhysicalDomain=network_engine_domain  SubClassName=ps_output  LeftPortType=input  RightPortType=output  PseudoPeriodic=off  Frequencies=[]  VectorFormat=1-D array  Unit=inherit  AffineConversion=off
  PS-Simulink Converter1 : nesl_utility/PS-Simulink Converter  PhysicalDomain=network_engine_domain  SubClassName=ps_output  LeftPortType=input  RightPortType=output  PseudoPeriodic=off  Frequencies=[]  VectorFormat=1-D array  Unit=inherit  AffineConversion=off
  PS-Simulink Converter2 : nesl_utility/PS-Simulink Converter  PhysicalDomain=network_engine_domain  SubClassName=ps_output  LeftPortType=input  RightPortType=output  PseudoPeriodic=off  Frequencies=[]  VectorFormat=1-D array  Unit=inherit  AffineConversion=off
  Sum : Sum  Inputs=|+-
  Sum1 : Sum  Inputs=|+-
  Sum2 : Sum  Inputs=|+-
  Voltage Sensor : fl_lib/Electrical/Electrical Sensors/Voltage Sensor
  Voltage Sensor1 : fl_lib/Electrical/Electrical Sensors/Voltage Sensor
  Voltage Sensor2 : fl_lib/Electrical/Electrical Sensors/Voltage Sensor
  va : PMIOPort  Side=Left
  vb : PMIOPort  Port=2  Side=Left
  vc : PMIOPort  Port=3  Side=Left
  tag scope: vabc_grid_A=global
  wires:
  Mux/1 -> [vabc_grid_A]
  Gain6/1 -> Mux/3
  Gain4/1 -> Mux/1
  Gain5/1 -> Mux/2
  PS-Simulink Converter/1 -> Sum/1, Sum1/2
  Sum/1 -> Gain4/1
  PS-Simulink Converter2/1 -> Sum2/1, Sum/2
  Sum1/1 -> Gain5/1
  PS-Simulink Converter1/1 -> Sum2/2, Sum1/1
  Sum2/1 -> Gain6/1
  connections:
  Voltage Sensor/LConn1 -- Voltage Sensor2/RConn2 -- va/RConn1
  vb/RConn1 -- Voltage Sensor1/LConn1 -- Voltage Sensor/RConn2
  Voltage Sensor/RConn1 -- PS-Simulink Converter/LConn1
  Voltage Sensor1/RConn1 -- PS-Simulink Converter1/LConn1
  Voltage Sensor1/RConn2 -- Voltage Sensor2/LConn1 -- vc/RConn1
  Voltage Sensor2/RConn1 -- PS-Simulink Converter2/LConn1

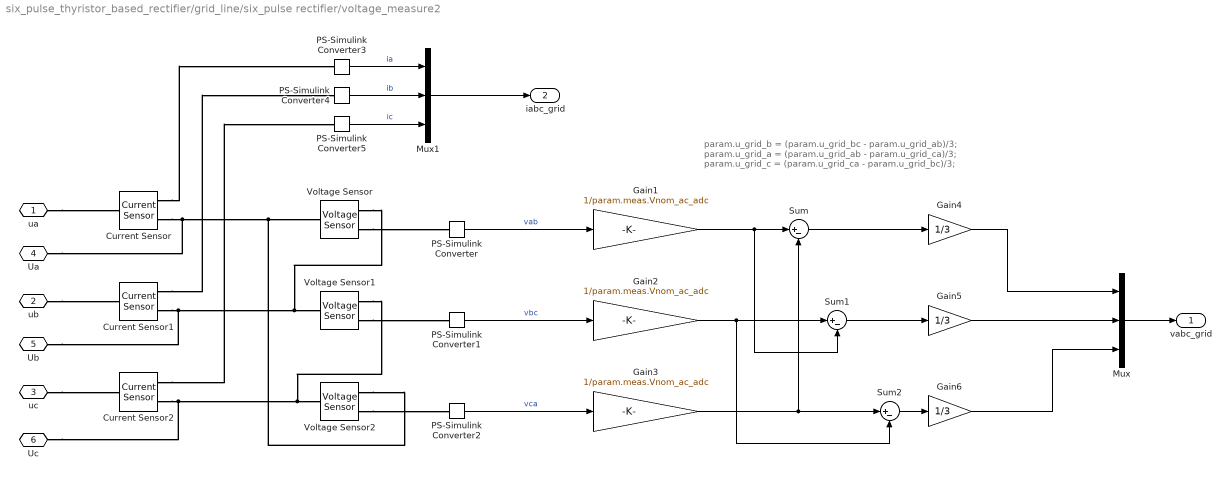
== system six_pulse_thyristor_based_rectifier/grid_line/six_pulse rectifier/voltage_measure2 ==
  note: param.u_grid_b = (param.u_grid_bc - param.u_grid_ab)/3;
      | 	param.u_grid_a = (param.u_grid_ab - param.u_grid_ca)/3;
      | 	param.u_grid_c = (param.u_grid_ca - param.u_grid_bc)/3;
  Current Sensor : fl_lib/Electrical/Electrical Sensors/Current Sensor
  Current Sensor1 : fl_lib/Electrical/Electrical Sensors/Current Sensor
  Current Sensor2 : fl_lib/Electrical/Electrical Sensors/Current Sensor
  Gain1 : Gain  Gain=1/param.meas.Vnom_ac_adc
  Gain2 : Gain  Gain=1/param.meas.Vnom_ac_adc
  Gain3 : Gain  Gain=1/param.meas.Vnom_ac_adc
  Gain4 : Gain  Gain=1/3
  Gain5 : Gain  Gain=1/3
  Gain6 : Gain  Gain=1/3
  Mux : Mux  Inputs=3
  Mux1 : Mux  Inputs=3
  PS-Simulink Converter : nesl_utility/PS-Simulink Converter  PhysicalDomain=network_engine_domain  SubClassName=ps_output  LeftPortType=input  RightPortType=output  PseudoPeriodic=off  Frequencies=[]  VectorFormat=1-D array  Unit=inherit  AffineConversion=off
  PS-Simulink Converter1 : nesl_utility/PS-Simulink Converter  PhysicalDomain=network_engine_domain  SubClassName=ps_output  LeftPortType=input  RightPortType=output  PseudoPeriodic=off  Frequencies=[]  VectorFormat=1-D array  Unit=inherit  AffineConversion=off
  PS-Simulink Converter2 : nesl_utility/PS-Simulink Converter  PhysicalDomain=network_engine_domain  SubClassName=ps_output  LeftPortType=input  RightPortType=output  PseudoPeriodic=off  Frequencies=[]  VectorFormat=1-D array  Unit=inherit  AffineConversion=off
  PS-Simulink Converter3 : nesl_utility/PS-Simulink Converter  PhysicalDomain=network_engine_domain  SubClassName=ps_output  LeftPortType=input  RightPortType=output  PseudoPeriodic=off  Frequencies=[]  VectorFormat=1-D array  Unit=A  AffineConversion=off
  PS-Simulink Converter4 : nesl_utility/PS-Simulink Converter  PhysicalDomain=network_engine_domain  SubClassName=ps_output  LeftPortType=input  RightPortType=output  PseudoPeriodic=off  Frequencies=[]  VectorFormat=1-D array  Unit=A  AffineConversion=off
  PS-Simulink Converter5 : nesl_utility/PS-Simulink Converter  PhysicalDomain=network_engine_domain  SubClassName=ps_output  LeftPortType=input  RightPortType=output  PseudoPeriodic=off  Frequencies=[]  VectorFormat=1-D array  Unit=A  AffineConversion=off
  Sum : Sum  Inputs=|+-
  Sum1 : Sum  Inputs=|+-
  Sum2 : Sum  Inputs=|+-
  Voltage Sensor : fl_lib/Electrical/Electrical Sensors/Voltage Sensor
  Voltage Sensor1 : fl_lib/Electrical/Electrical Sensors/Voltage Sensor
  Voltage Sensor2 : fl_lib/Electrical/Electrical Sensors/Voltage Sensor
  ua : PMIOPort  Side=Left
  ub : PMIOPort  Port=2  Side=Left
  uc : PMIOPort  Port=3  Side=Left
  Ua : PMIOPort  Port=4  Side=Right
  Ub : PMIOPort  Port=5  Side=Right
  Uc : PMIOPort  Port=6  Side=Right
  vabc_grid : Outport
  iabc_grid : Outport  Port=2
  wires:
  PS-Simulink Converter1/1 -> Gain2/1  "vbc"
  PS-Simulink Converter2/1 -> Gain3/1  "vca"
  PS-Simulink Converter/1 -> Gain1/1  "vab"
  Mux/1 -> vabc_grid/1
  Gain1/1 -> Sum1/2, Sum/1
  Gain3/1 -> Sum2/1, Sum/2
  Sum/1 -> Gain4/1
  Sum1/1 -> Gain5/1
  Sum2/1 -> Gain6/1
  Gain2/1 -> Sum2/2, Sum1/1
  Gain4/1 -> Mux/1
  Gain5/1 -> Mux/2
  Gain6/1 -> Mux/3
  Mux1/1 -> iabc_grid/1
  PS-Simulink Converter4/1 -> Mux1/2  "ib"
  PS-Simulink Converter3/1 -> Mux1/1  "ia"
  PS-Simulink Converter5/1 -> Mux1/3  "ic"
  connections:
  Voltage Sensor/RConn2 -- Ub/RConn1 -- Current Sensor1/RConn2 -- Voltage Sensor1/LConn1
  Voltage Sensor2/RConn2 -- Ua/RConn1 -- Current Sensor/RConn2 -- Voltage Sensor/LConn1
  Voltage Sensor/RConn1 -- PS-Simulink Converter/LConn1
  Voltage Sensor2/RConn1 -- PS-Simulink Converter2/LConn1
  Voltage Sensor1/RConn2 -- Uc/RConn1 -- Current Sensor2/RConn2 -- Voltage Sensor2/LConn1
  Voltage Sensor1/RConn1 -- PS-Simulink Converter1/LConn1
  ua/RConn1 -- Current Sensor/LConn1
  ub/RConn1 -- Current Sensor1/LConn1
  uc/RConn1 -- Current Sensor2/LConn1
  Current Sensor/RConn1 -- PS-Simulink Converter3/LConn1
  Current Sensor1/RConn1 -- PS-Simulink Converter4/LConn1
  Current Sensor2/RConn1 -- PS-Simulink Converter5/LConn1

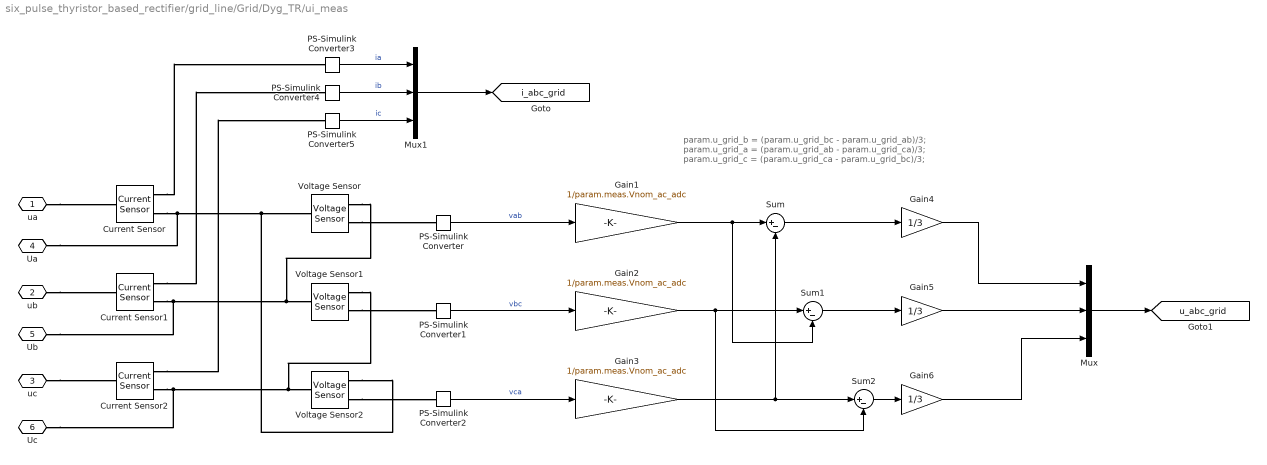
== system six_pulse_thyristor_based_rectifier/grid_line/Grid/Dyg_TR/ui_meas ==
  note: param.u_grid_b = (param.u_grid_bc - param.u_grid_ab)/3;
      | 	param.u_grid_a = (param.u_grid_ab - param.u_grid_ca)/3;
      | 	param.u_grid_c = (param.u_grid_ca - param.u_grid_bc)/3;
  Current Sensor : fl_lib/Electrical/Electrical Sensors/Current Sensor
  Current Sensor1 : fl_lib/Electrical/Electrical Sensors/Current Sensor
  Current Sensor2 : fl_lib/Electrical/Electrical Sensors/Current Sensor
  Gain1 : Gain  Gain=1/param.meas.Vnom_ac_adc
  Gain2 : Gain  Gain=1/param.meas.Vnom_ac_adc
  Gain3 : Gain  Gain=1/param.meas.Vnom_ac_adc
  Gain4 : Gain  Gain=1/3
  Gain5 : Gain  Gain=1/3
  Gain6 : Gain  Gain=1/3
  Mux : Mux  Inputs=3
  Mux1 : Mux  Inputs=3
  PS-Simulink Converter : nesl_utility/PS-Simulink Converter  PhysicalDomain=network_engine_domain  SubClassName=ps_output  LeftPortType=input  RightPortType=output  PseudoPeriodic=off  Frequencies=[]  VectorFormat=1-D array  Unit=inherit  AffineConversion=off
  PS-Simulink Converter1 : nesl_utility/PS-Simulink Converter  PhysicalDomain=network_engine_domain  SubClassName=ps_output  LeftPortType=input  RightPortType=output  PseudoPeriodic=off  Frequencies=[]  VectorFormat=1-D array  Unit=inherit  AffineConversion=off
  PS-Simulink Converter2 : nesl_utility/PS-Simulink Converter  PhysicalDomain=network_engine_domain  SubClassName=ps_output  LeftPortType=input  RightPortType=output  PseudoPeriodic=off  Frequencies=[]  VectorFormat=1-D array  Unit=inherit  AffineConversion=off
  PS-Simulink Converter3 : nesl_utility/PS-Simulink Converter  PhysicalDomain=network_engine_domain  SubClassName=ps_output  LeftPortType=input  RightPortType=output  PseudoPeriodic=off  Frequencies=[]  VectorFormat=1-D array  Unit=A  AffineConversion=off
  PS-Simulink Converter4 : nesl_utility/PS-Simulink Converter  PhysicalDomain=network_engine_domain  SubClassName=ps_output  LeftPortType=input  RightPortType=output  PseudoPeriodic=off  Frequencies=[]  VectorFormat=1-D array  Unit=A  AffineConversion=off
  PS-Simulink Converter5 : nesl_utility/PS-Simulink Converter  PhysicalDomain=network_engine_domain  SubClassName=ps_output  LeftPortType=input  RightPortType=output  PseudoPeriodic=off  Frequencies=[]  VectorFormat=1-D array  Unit=A  AffineConversion=off
  Sum : Sum  Inputs=|+-
  Sum1 : Sum  Inputs=|+-
  Sum2 : Sum  Inputs=|+-
  Voltage Sensor : fl_lib/Electrical/Electrical Sensors/Voltage Sensor
  Voltage Sensor1 : fl_lib/Electrical/Electrical Sensors/Voltage Sensor
  Voltage Sensor2 : fl_lib/Electrical/Electrical Sensors/Voltage Sensor
  ua : PMIOPort  Side=Left
  ub : PMIOPort  Port=2  Side=Left
  uc : PMIOPort  Port=3  Side=Left
  Ua : PMIOPort  Port=4  Side=Right
  Ub : PMIOPort  Port=5  Side=Right
  Uc : PMIOPort  Port=6  Side=Right
  tag scope: i_abc_grid=global, u_abc_grid=global
  wires:
  PS-Simulink Converter5/1 -> Mux1/3  "ic"
  PS-Simulink Converter3/1 -> Mux1/1  "ia"
  PS-Simulink Converter4/1 -> Mux1/2  "ib"
  Gain6/1 -> Mux/3
  Gain5/1 -> Mux/2
  Gain4/1 -> Mux/1
  Gain2/1 -> Sum1/1, Sum2/2
  Sum2/1 -> Gain6/1
  Sum1/1 -> Gain5/1
  Sum/1 -> Gain4/1
  Gain3/1 -> Sum/2, Sum2/1
  Gain1/1 -> Sum/1, Sum1/2
  PS-Simulink Converter/1 -> Gain1/1  "vab"
  PS-Simulink Converter2/1 -> Gain3/1  "vca"
  PS-Simulink Converter1/1 -> Gain2/1  "vbc"
  Mux1/1 -> [i_abc_grid]
  Mux/1 -> [u_abc_grid]
  connections:
  Current Sensor2/RConn1 -- PS-Simulink Converter5/LConn1
  Current Sensor1/RConn1 -- PS-Simulink Converter4/LConn1
  Current Sensor/RConn1 -- PS-Simulink Converter3/LConn1
  uc/RConn1 -- Current Sensor2/LConn1
  ub/RConn1 -- Current Sensor1/LConn1
  ua/RConn1 -- Current Sensor/LConn1
  Voltage Sensor1/RConn1 -- PS-Simulink Converter1/LConn1
  Uc/RConn1 -- Current Sensor2/RConn2 -- Voltage Sensor1/RConn2 -- Voltage Sensor2/LConn1
  Voltage Sensor2/RConn1 -- PS-Simulink Converter2/LConn1
  Voltage Sensor/RConn1 -- PS-Simulink Converter/LConn1
  Ua/RConn1 -- Current Sensor/RConn2 -- Voltage Sensor2/RConn2 -- Voltage Sensor/LConn1
  Ub/RConn1 -- Current Sensor1/RConn2 -- Voltage Sensor/RConn2 -- Voltage Sensor1/LConn1

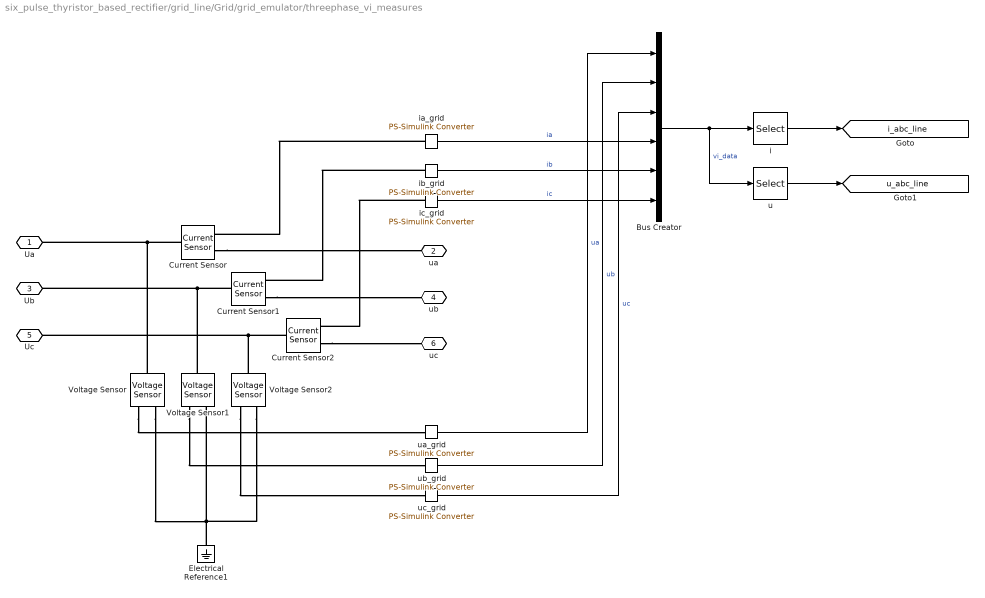
== system six_pulse_thyristor_based_rectifier/grid_line/Grid/grid_emulator/threephase_vi_measures ==
  Bus Creator : BusCreator  Inputs=6
  Current Sensor : fl_lib/Electrical/Electrical Sensors/Current Sensor
  Current Sensor1 : fl_lib/Electrical/Electrical Sensors/Current Sensor
  Current Sensor2 : fl_lib/Electrical/Electrical Sensors/Current Sensor
  Electrical Reference1 : fl_lib/Electrical/Electrical Elements/Electrical Reference
  Voltage Sensor : fl_lib/Electrical/Electrical Sensors/Voltage Sensor
  Voltage Sensor1 : fl_lib/Electrical/Electrical Sensors/Voltage Sensor
  Voltage Sensor2 : fl_lib/Electrical/Electrical Sensors/Voltage Sensor
  i : Selector  InputPortWidth=6  IndexOptions=Index vector (dialog)  Indices=[4 5 6]  OutputSizes=1  RuntimeRangeChecks=off
  ia_grid : nesl_utility/PS-Simulink Converter  PhysicalDomain=network_engine_domain  SubClassName=ps_output  LeftPortType=input  RightPortType=output  PseudoPeriodic=off  Frequencies=[]  VectorFormat=1-D array  Unit=A  AffineConversion=off
  ib_grid : nesl_utility/PS-Simulink Converter  PhysicalDomain=network_engine_domain  SubClassName=ps_output  LeftPortType=input  RightPortType=output  PseudoPeriodic=off  Frequencies=[]  VectorFormat=1-D array  Unit=A  AffineConversion=off
  ic_grid : nesl_utility/PS-Simulink Converter  PhysicalDomain=network_engine_domain  SubClassName=ps_output  LeftPortType=input  RightPortType=output  PseudoPeriodic=off  Frequencies=[]  VectorFormat=1-D array  Unit=A  AffineConversion=off
  u : Selector  InputPortWidth=6  IndexOptions=Index vector (dialog)  Indices=[1 2 3]  OutputSizes=1  RuntimeRangeChecks=off
  ua_grid : nesl_utility/PS-Simulink Converter  PhysicalDomain=network_engine_domain  SubClassName=ps_output  LeftPortType=input  RightPortType=output  PseudoPeriodic=off  Frequencies=[]  VectorFormat=1-D array  Unit=V  AffineConversion=off
  ub_grid : nesl_utility/PS-Simulink Converter  PhysicalDomain=network_engine_domain  SubClassName=ps_output  LeftPortType=input  RightPortType=output  PseudoPeriodic=off  Frequencies=[]  VectorFormat=1-D array  Unit=V  AffineConversion=off
  uc_grid : nesl_utility/PS-Simulink Converter  PhysicalDomain=network_engine_domain  SubClassName=ps_output  LeftPortType=input  RightPortType=output  PseudoPeriodic=off  Frequencies=[]  VectorFormat=1-D array  Unit=V  AffineConversion=off
  Ua : PMIOPort  Side=Left
  ua : PMIOPort  Port=2  Side=Right
  Ub : PMIOPort  Port=3  Side=Left
  ub : PMIOPort  Port=4  Side=Right
  Uc : PMIOPort  Port=5  Side=Left
  uc : PMIOPort  Port=6  Side=Right
  tag scope: i_abc_line=global, u_abc_line=global
  wires:
  Bus Creator/1 -> i/1, u/1  "vi_data"
  ib_grid/1 -> Bus Creator/5  "ib"
  ia_grid/1 -> Bus Creator/4  "ia"
  ic_grid/1 -> Bus Creator/6  "ic"
  ua_grid/1 -> Bus Creator/1  "ua"
  ub_grid/1 -> Bus Creator/2  "ub"
  uc_grid/1 -> Bus Creator/3  "uc"
  i/1 -> [i_abc_line]
  u/1 -> [u_abc_line]
  connections:
  Current Sensor1/LConn1 -- Ub/RConn1 -- Voltage Sensor1/LConn1
  Electrical Reference1/LConn1 -- Voltage Sensor/RConn2 -- Voltage Sensor2/RConn2 -- Voltage Sensor1/RConn2
  Voltage Sensor/RConn1 -- ua_grid/LConn1
  Current Sensor/RConn2 -- ua/RConn1
  Voltage Sensor1/RConn1 -- ub_grid/LConn1
  Voltage Sensor2/LConn1 -- Current Sensor2/LConn1 -- Uc/RConn1
  Current Sensor/LConn1 -- Ua/RConn1 -- Voltage Sensor/LConn1
  Current Sensor1/RConn2 -- ub/RConn1
  Voltage Sensor2/RConn1 -- uc_grid/LConn1
  ib_grid/LConn1 -- Current Sensor1/RConn1
  ia_grid/LConn1 -- Current Sensor/RConn1
  ic_grid/LConn1 -- Current Sensor2/RConn1
  Current Sensor2/RConn2 -- uc/RConn1

== system six_pulse_thyristor_based_rectifier/grid_line/Grid/pwr-measurement/THD ==
  Constant : Constant  Value=1/param.glb_time.tc
  Constant1 : Constant  Value=25
  Constant2 : Constant  Value=200e-3/param.glb_time.tc
  Constant3 : Constant  Value=10e-3/param.glb_time.tc
  Data Type Conversion : DataTypeConversion  OutDataTypeStr=int32  SaturateOnIntegerOverflow=off  RndMeth=Floor
  Data Type Conversion1 : DataTypeConversion  OutDataTypeStr=int32  SaturateOnIntegerOverflow=off  RndMeth=Floor
  Data Type Conversion2 : DataTypeConversion  OutDataTypeStr=int32  SaturateOnIntegerOverflow=off  RndMeth=Floor
  Selector : Selector  InputPortWidth=3  IndexOptions=Index vector (dialog)  Indices=1  OutputSizes=1
  THDi : Scope  NumInputPorts=3
      settings: ActiveDisplayYMinimum=-13.665284988065604  ActiveDisplayYMaximum=122.98756489259047  DataLoggingVariableName=ScopeData14
  thd : MATLAB Function  TreatAsAtomicUnit=on  SystemSampleTime=param.glb_time.tc
  wires:
  Constant3/1 -> Data Type Conversion1/1
  Constant2/1 -> Data Type Conversion/1
  thd/1(thd_pct) -> THDi/1
  Constant1/1 -> Data Type Conversion2/1
  thd/2(f1) -> THDi/2
  thd/3(valid) -> THDi/3
  Constant/1 -> thd/2(fs)
  Data Type Conversion/1 -> thd/4(N)
  Data Type Conversion1/1 -> thd/5(Nupd)
  Data Type Conversion2/1 -> thd/3(nHarm)
  [i_abc_line] -> Selector/1
  Selector/1 -> thd/1(u)
